simulink model "DRLHevIps"  (R2025b)
settings: Solver=ode23tb  StartTime=0  StopTime=stop_time+1  FixedStep=ts  RelTol=1e-3  AbsTol=1e-4
model workspace (MAT data in the model file):
  BattChrgMax : Simulink.Parameter (value not decoded)
  BattDischrgMax : Simulink.Parameter (value not decoded)
  BrkPrsMax : Simulink.Parameter (value not decoded)
  DiffRatio : Simulink.Parameter (value not decoded)
  EVSpdLmt : Simulink.Parameter (value not decoded)
  EngIdle : Simulink.Parameter (value not decoded)
  EngPwr : Simulink.Parameter (value not decoded)
  EngSpd : Simulink.Parameter (value not decoded)
  EngTrq : Simulink.Parameter (value not decoded)
  EngTrqWhl : Simulink.Parameter (value not decoded)
  GenMapEff : Simulink.Parameter (value not decoded)
  GenMapSpdIndex : Simulink.Parameter (value not decoded)
  GenMapTrqIndex : Simulink.Parameter (value not decoded)
  GenPwrMax : Simulink.Parameter (value not decoded)
  GenSpd : Simulink.Parameter (value not decoded)
  GenTrq : Simulink.Parameter (value not decoded)
  GenTrqMax : Simulink.Parameter (value not decoded)
  MotMapEff : Simulink.Parameter (value not decoded)
  MotMapSpdIndex : Simulink.Parameter (value not decoded)
  MotMapTrqIndex : Simulink.Parameter (value not decoded)
  MotPwr : Simulink.Parameter (value not decoded)
  MotSpd : Simulink.Parameter (value not decoded)
  MotTrq : Simulink.Parameter (value not decoded)
  Ndiff : Simulink.Parameter (value not decoded)
  Nr1 : Simulink.Parameter (value not decoded)
  Nr2 : Simulink.Parameter (value not decoded)
  Ns1 : Simulink.Parameter (value not decoded)
  Ns2 : Simulink.Parameter (value not decoded)
  NsysWhl : Simulink.Parameter (value not decoded)
  SOCChrgFactor : Simulink.Parameter (value not decoded)
  SOCerr : Simulink.Parameter (value not decoded)
  SOCmax : Simulink.Parameter (value not decoded)
  SOCmin : Simulink.Parameter (value not decoded)
  SOCtarget : Simulink.Parameter (value not decoded)
  SysTrqWhl : Simulink.Parameter (value not decoded)
  k : Simulink.Parameter (value not decoded)
values from neighbouring files (symbols this model uses):
  cyc_time = WLTC(:,1)    [mdlrun_time_DG.m]
  cyc_vel = WLTC(:,2)    [mdlrun_time_DG.m]
  en_actsmo = 1    [mdlrun_time_DG.m]
  en_elec = 1    [mdlrun_time_DG.m]
  en_gas = 1    [mdlrun_time_DG.m]
  en_SOCpen = 1    [mdlrun_time_DG.m]
  k_actsmo = 5e-2    (= 0.05)    [mdlrun_time_DG.m]
  k_elec = 1    [mdlrun_time_DG.m]
  k_gas = 1    [mdlrun_time_DG.m]
  k_SOCpen = 1.2    [mdlrun_time_DG.m]
  obs_max = 1e4*[0.0020, 0.0090, 0.0100, 0.0100, 8.4000, 0.0100,                0.0056, 0.1011, 2.8000,      0, 0.0001, 0.0132,                0.0740, 2.6065, 0.0339, 0.0949, 0.0117, 2.4444]    [mdlrun_time_DG.m]
  obs_min = 1e4*[0.0010, 0.0070,      0,      0, 0.8400,      0,                     0, -0.0005,     0, -2.8000,     0, -0.0032               -0.0694, -2.7092, -0.0030,    0, -0.0001, -2.7647]    [mdlrun_time_DG.m]
  Price_elec = 1    [mdlrun_time_DG.m]
  Price_gas = 7.14    [mdlrun_time_DG.m]
  rho_gas = 0.739    [mdlrun_time_DG.m]
  stop_time = cyc_time(end)    [mdlrun_time_DG.m]
  ts = 1    [mdlrun_time_DG.m]
symbols that are objects in the model workspace (value not decoded): BattChrgMax, BattDischrgMax, BrkPrsMax, DiffRatio, EngIdle, EngPwr, EngSpd, EngTrq, EngTrqWhl, EVSpdLmt, GenMapSpdIndex, GenMapTrqIndex, GenPwrMax, GenSpd, GenTrq, GenTrqMax, k, MotMapSpdIndex, MotMapTrqIndex, MotPwr, MotSpd, MotTrq, Ndiff, Nr1, Nr2, Ns1, Ns2, NsysWhl, SOCChrgFactor, SOCerr, SOCmin, SOCtarget, SysTrqWhl
undefined symbols (not defined in the file or in its folder): n_ool, T_ool
libraries: simulink x29, autolibutils x6, slpidlib x2, rllib x2, SignalEditorBlockLib x1, autolibshared x1, autolibhevctrlrcommon x1
(part 4 of 4)

== system DRLHevIps/xCU/xCU/VCU/Rule_Based_DataGen/Subsystem ==
  note: 4 brakes*(mu*pi*Ba^2*Rm*Npads/4)*P
  note: T / 4 brakes*(mu*pi*Ba^2*Rm*Npads/4)
  BattSoc : Inport
  VehSpd : Inport  Port=2
  MotSpd : Inport  Port=3
  "BrkPrsReq " : Inport  Port=4
  ChrgLmt : Lookup_n-D  NumberOfTableDimensions=1  BreakpointsForDimension1=[0:10:100]  Table=[1 1 1 1 1 1 1 1 0.7 0.35 0]  ExtrapMethod=Clip  UseLastTableValue=on  InternalRulePriority=Speed  RndMeth=Simplest
  Constant : Constant  Value=4*(0.2*pi*0.05^2*0.1778*2/4)
  Constant1 : Constant  Value=4*(0.2*pi*0.05^2*0.1778*2/4)
  Gain : Gain  Gain=-1
  MaxMotTrqVsSpd : Lookup_n-D  NumberOfTableDimensions=1  BreakpointsForDimension1=MotSpd  Table=MotTrq  ExtrapMethod=Clip  UseLastTableValue=on  InternalRulePriority=Speed  OutDataTypeStr=Inherit: Inherit from 'Table data'  RndMeth=Simplest
  MinMax : MinMax  Inputs=2
  MotTrqReflectedToWheels : Gain  Gain=(Nr2/Ns2)*Ndiff
  Negative 5 : Saturate  UpperLimit=inf  LowerLimit=0
  Product1 : Product
  Product2 : Product
  Product3 : Product
  Product4 : Product  Inputs=*/
  RegenBrakingCutoff : Lookup_n-D  NumberOfTableDimensions=1  BreakpointsForDimension1=[2.2 4.5]  Table=[0 1]  ExtrapMethod=Clip  UseLastTableValue=on  InternalRulePriority=Speed  RndMeth=Simplest
  Subtract : Sum  Inputs=+-
  WhlTrqReflectedToMot : Gain  Gain=1/((Nr2/Ns2)*Ndiff)
  rads_to_rpm : Gain  Gain=30/pi
  " MotTrqCmdRegen" : Outport  VectorParamsAs1DForOutWhenUnconnected=off
  " BrkCmd" : Outport  Port=2  VectorParamsAs1DForOutWhenUnconnected=off
  wires:
  VehSpd/1 -> RegenBrakingCutoff/1
  Subtract/1 -> Negative 5/1
  Product4/1 -> " BrkCmd"/1
  RegenBrakingCutoff/1 -> Product1/1
  "BrkPrsReq "/1 -> Product2/1  "BrkPrsReq"
  Negative 5/1 -> Product4/1  "BrkTrqFric"
  MaxMotTrqVsSpd/1 -> MotTrqReflectedToWheels/1  "MotTrqMax"
  MotSpd/1 -> rads_to_rpm/1
  MinMax/1 -> Product3/1  "min"
  Product2/1 -> MinMax/1, Subtract/1  "BrkTrqReqTotal"
  rads_to_rpm/1 -> MaxMotTrqVsSpd/1
  Gain/1 -> " MotTrqCmdRegen"/1  "MotTrqCmdRegen"
  Product1/1 -> Product3/2  "RegenFactor"
  Product3/1 -> WhlTrqReflectedToMot/1, Subtract/2  "MotTrqRegenWhl"
  WhlTrqReflectedToMot/1 -> Gain/1
  ChrgLmt/1 -> Product1/2
  BattSoc/1 -> ChrgLmt/1
  Constant/1 -> Product2/2
  MotTrqReflectedToWheels/1 -> MinMax/2  "MotTrqMaxWhls"
  Constant1/1 -> Product4/2

== system DRLHevIps/xCU/xCU/VCU/DRL_Based2_0/Motor Torque Arbitration and Power Management/Power Management ==
  BattPwrDischrgLmt : Inport
  GenPwrElec : Inport  Port=2
  BattPwrChrgLmt : Inport  Port=3
  MotSpd : Inport  Port=4
  MotTrqCmd : Inport  Port=5
  Check Within Limits : Subsystem
  ElecToMechPwr : Product  Inputs=*/
  Mech to Elec Power Estimate : Subsystem
  MechPwrToTrq : Product  Inputs=*/
  Saturation1 : Saturate  UpperLimit=inf  LowerLimit=0
  Saturation2 : Saturate  UpperLimit=0  LowerLimit=-inf
  Sum : Sum  Inputs=+-
  Sum4 : Sum  Inputs=-+
  Switch : Switch  Criteria=u2 > Threshold  SaturateOnIntegerOverflow=off  InputSameDT=off
  Torque Limit : Subsystem
  div0protect - poly : autolibutils/div0protect - poly  thresh=2  ZeroCross1=off  aMode=aMode
  MotTrqLim : Outport  VectorParamsAs1DForOutWhenUnconnected=off
  wires:
  Check Within Limits/1(InLimit) -> Switch/2
  Switch/1 -> Torque Limit/1(MotTrq)
  Check Within Limits/2(y) -> ElecToMechPwr/1
  Saturation2/1 -> Check Within Limits/3(lo)
  Mech to Elec Power Estimate/1(MotPwrElecReq) -> Check Within Limits/2(u)
  Saturation1/1 -> Check Within Limits/1(up)
  Torque Limit/1(MotTrqCmd) -> MotTrqLim/1
  MechPwrToTrq/1 -> Switch/3
  ElecToMechPwr/1 -> MechPwrToTrq/1
  Mech to Elec Power Estimate/2(eff2k) -> ElecToMechPwr/2
  div0protect - poly/1 -> MechPwrToTrq/2
  MotTrqCmd/1 -> Mech to Elec Power Estimate/1(MotTrqCmd), Switch/1
  MotSpd/1 -> Mech to Elec Power Estimate/2(MotSpd), div0protect - poly/1, Torque Limit/2(MotSpd)
  BattPwrDischrgLmt/1 -> Sum/1
  GenPwrElec/1 -> Sum4/1, Sum/2
  Sum/1 -> Saturation1/1
  Sum4/1 -> Saturation2/1
  BattPwrChrgLmt/1 -> Sum4/2

== system DRLHevIps/xCU/xCU/VCU/Rule_Based/Motor Torque Arbitration and Power Management/Power Management ==
  BattPwrDischrgLmt : Inport
  GenPwrElec : Inport  Port=2
  BattPwrChrgLmt : Inport  Port=3
  MotSpd : Inport  Port=4
  MotTrqCmd : Inport  Port=5
  Check Within Limits : Subsystem
  ElecToMechPwr : Product  Inputs=*/
  Mech to Elec Power Estimate : Subsystem
  MechPwrToTrq : Product  Inputs=*/
  Saturation1 : Saturate  UpperLimit=inf  LowerLimit=0
  Saturation2 : Saturate  UpperLimit=0  LowerLimit=-inf
  Sum : Sum  Inputs=+-
  Sum4 : Sum  Inputs=-+
  Switch : Switch  Criteria=u2 > Threshold  SaturateOnIntegerOverflow=off  InputSameDT=off
  Torque Limit : Subsystem
  div0protect - poly : autolibutils/div0protect - poly  thresh=2  ZeroCross1=off  aMode=aMode
  MotTrqLim : Outport  VectorParamsAs1DForOutWhenUnconnected=off
  wires:
  BattPwrChrgLmt/1 -> Sum4/2
  Sum4/1 -> Saturation2/1
  Sum/1 -> Saturation1/1
  GenPwrElec/1 -> Sum/2, Sum4/1
  BattPwrDischrgLmt/1 -> Sum/1
  MotSpd/1 -> Torque Limit/2(MotSpd), div0protect - poly/1, Mech to Elec Power Estimate/2(MotSpd)
  MotTrqCmd/1 -> Switch/1, Mech to Elec Power Estimate/1(MotTrqCmd)
  div0protect - poly/1 -> MechPwrToTrq/2
  Mech to Elec Power Estimate/2(eff2k) -> ElecToMechPwr/2
  ElecToMechPwr/1 -> MechPwrToTrq/1
  MechPwrToTrq/1 -> Switch/3
  Torque Limit/1(MotTrqCmd) -> MotTrqLim/1
  Saturation1/1 -> Check Within Limits/1(up)
  Mech to Elec Power Estimate/1(MotPwrElecReq) -> Check Within Limits/2(u)
  Saturation2/1 -> Check Within Limits/3(lo)
  Check Within Limits/2(y) -> ElecToMechPwr/1
  Switch/1 -> Torque Limit/1(MotTrq)
  Check Within Limits/1(InLimit) -> Switch/2

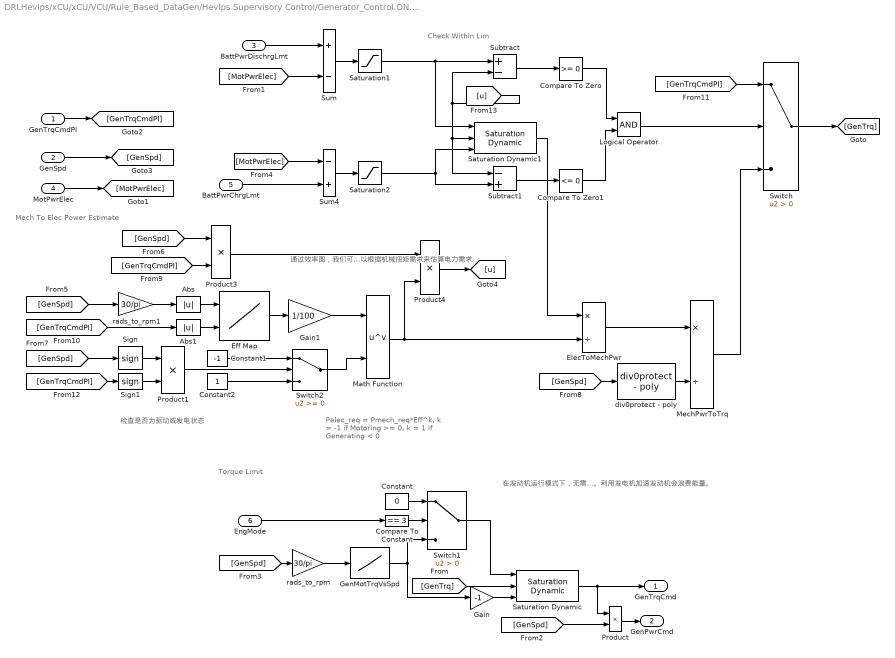
== system DRLHevIps/xCU/xCU/VCU/Rule_Based_DataGen/HevIps Supervisory Control/Generator_Control.ON.GenControl/Power Management ==
  note: Check Within Lim
  note: Mech To Elec Power Estimate
  note: Torque Limit
  note: 在发动机运行模式下，无需保持发电机扭矩大于零，因为发电机通过制动发动机来维持所需速度。利用发电机加速发动机会浪费能量。
  note: 检查是否为驱动或发电状态
  note: 通过效率图，我们可以根据机械扭矩需求来估算电力需求。
  note: Pelec_req = Pmech_req*Eff^k,
      | k = -1 if Motoring >= 0,
      | k = 1 if Generating < 0
  GenTrqCmdPI : Inport
  GenSpd : Inport  Port=2
  BattPwrDischrgLmt : Inport  Port=3
  MotPwrElec : Inport  Port=4
  BattPwrChrgLmt : Inport  Port=5
  EngMode : Inport  Port=6
  Abs : Abs  SaturateOnIntegerOverflow=off
  Abs1 : Abs  SaturateOnIntegerOverflow=off
  Compare To Constant : simulink/Logic and Bit Operations/Compare To Constant  relop===  const=3  OutDataTypeStr=boolean
  Compare To Zero : simulink/Logic and Bit Operations/Compare To Zero  relop=>=  OutDataTypeStr=boolean
  Compare To Zero1 : simulink/Logic and Bit Operations/Compare To Zero  relop=<=  OutDataTypeStr=boolean
  Constant : Constant  Value=0
  Constant1 : Constant  Value=-1  SampleTime=-1
  Constant2 : Constant  SampleTime=-1
  Eff Map : Lookup_n-D  BreakpointsForDimension1=GenMapSpdIndex  BreakpointsForDimension2=GenMapTrqIndex  Table=GenMapEff'  ExtrapMethod=Clip  UseLastTableValue=on  InternalRulePriority=Speed  OutDataTypeStr=Inherit: Inherit from 'Table data'  RndMeth=Simplest
      settings: InputPortMap=u0,u1
  ElecToMechPwr : Product  Inputs=*/
  Gain : Gain  Gain=-1
  Gain1 : Gain  Gain=1/100
  GenMotTrqVsSpd : Lookup_n-D  NumberOfTableDimensions=1  BreakpointsForDimension1=GenSpd  Table=GenTrq  ExtrapMethod=Clip  UseLastTableValue=on  InternalRulePriority=Speed  OutDataTypeStr=Inherit: Inherit from 'Table data'  RndMeth=Simplest
  Logical Operator : Logic  AllPortsSameDT=off  OutDataTypeStr=boolean
  Math Function : Math  Operator=pow  SignedPower=on  OutputSignalType=real
  MechPwrToTrq : Product  Inputs=*/
  Product{,1,3..4} (4 alike) : Product
  Saturation Dynamic : simulink/Discontinuities/Saturation Dynamic  OutMin=[]  OutMax=[]  OutDataTypeStr=Inherit: Same as second input  OutDataType=fixdt(1, 16)  OutScaling=2^-10  DoSatur=off
  Saturation Dynamic1 : simulink/Discontinuities/Saturation Dynamic  OutMin=[]  OutMax=[]  OutDataTypeStr=Inherit: Same as second input  OutDataType=fixdt(1, 16)  OutScaling=2^-10  DoSatur=off
  Saturation1 : Saturate  UpperLimit=inf  LowerLimit=0
  Saturation2 : Saturate  UpperLimit=0  LowerLimit=-inf
  Sign : Signum
  Sign1 : Signum
  Subtract : Sum  Inputs=+-
  Subtract1 : Sum  Inputs=-+
  Sum : Sum  Inputs=+-
  Sum4 : Sum  Inputs=-+
  Switch : Switch  Criteria=u2 > Threshold  SaturateOnIntegerOverflow=off  InputSameDT=off
  Switch1 : Switch  Criteria=u2 > Threshold  SaturateOnIntegerOverflow=off  InputSameDT=off
  Switch2 : Switch  SaturateOnIntegerOverflow=off  InputSameDT=off
  div0protect - poly : autolibutils/div0protect - poly  thresh=2  ZeroCross1=off  aMode=aMode
  rads_to_rpm : Gain  Gain=30/pi
  rads_to_rpm1 : Gain  Gain=30/pi
  GenTrqCmd : Outport  VectorParamsAs1DForOutWhenUnconnected=off
  GenPwrCmd : Outport  Port=2  VectorParamsAs1DForOutWhenUnconnected=off
  wires:
  Logical Operator/1 -> Switch/2
  Switch/1 -> [GenTrq]
  Product/1 -> GenPwrCmd/1
  MechPwrToTrq/1 -> Switch/3
  Saturation Dynamic/1 -> Product/1, GenTrqCmd/1
  Math Function/1 -> Product4/2, ElecToMechPwr/2
  Saturation Dynamic1/1 -> ElecToMechPwr/1
  div0protect - poly/1 -> MechPwrToTrq/2
  ElecToMechPwr/1 -> MechPwrToTrq/1
  BattPwrDischrgLmt/1 -> Sum/1
  MotPwrElec/1 -> [MotPwrElec]
  Sum/1 -> Saturation1/1
  Sum4/1 -> Saturation2/1
  BattPwrChrgLmt/1 -> Sum4/2
  [GenSpd] -> Product/2
  rads_to_rpm/1 -> GenMotTrqVsSpd/1
  Constant/1 -> Switch1/1
  GenMotTrqVsSpd/1 -> Gain/1, Switch1/3
  Gain/1 -> Saturation Dynamic/3
  [GenTrq] -> Saturation Dynamic/2
  [GenSpd] -> rads_to_rpm/1
  EngMode/1 -> Compare To Constant/1
  Compare To Constant/1 -> Switch1/2
  Switch1/1 -> Saturation Dynamic/1
  Product3/1 -> Product4/1
  Switch2/1 -> Math Function/2
  Constant1/1 -> Switch2/1
  Constant2/1 -> Switch2/3
  Eff Map/1 -> Gain1/1
  GenTrqCmdPI/1 -> [GenTrqCmdPI]
  Abs/1 -> Eff Map/1
  Gain1/1 -> Math Function/1
  Abs1/1 -> Eff Map/2
  rads_to_rpm1/1 -> Abs/1
  Product1/1 -> Switch2/2
  Sign/1 -> Product1/1
  Sign1/1 -> Product1/2
  GenSpd/1 -> [GenSpd]
  [MotPwrElec] -> Sum/2
  [MotPwrElec] -> Sum4/1
  [GenSpd] -> Product3/1
  [GenSpd] -> rads_to_rpm1/1
  [GenSpd] -> Sign/1
  [GenSpd] -> div0protect - poly/1
  [GenTrqCmdPI] -> Product3/2
  [GenTrqCmdPI] -> Abs1/1
  [GenTrqCmdPI] -> Switch/1
  [GenTrqCmdPI] -> Sign1/1
  Product4/1 -> [u]
  Saturation2/1 -> Subtract1/2, Saturation Dynamic1/3
  Saturation1/1 -> Subtract/1, Saturation Dynamic1/1
  [u] -> Saturation Dynamic1/2, Subtract1/1, Subtract/2
  Subtract/1 -> Compare To Zero/1
  Subtract1/1 -> Compare To Zero1/1
  Compare To Zero/1 -> Logical Operator/1
  Compare To Zero1/1 -> Logical Operator/2

== system DRLHevIps/xCU/xCU/VCU/Rule_Based_DataGen/Motor Torque Arbitration and Power Management/Power Management ==
  BattPwrDischrgLmt : Inport
  GenPwrElec : Inport  Port=2
  BattPwrChrgLmt : Inport  Port=3
  MotSpd : Inport  Port=4
  MotTrqCmd : Inport  Port=5
  Check Within Limits : Subsystem
  ElecToMechPwr : Product  Inputs=*/
  Mech to Elec Power Estimate : Subsystem
  MechPwrToTrq : Product  Inputs=*/
  Saturation1 : Saturate  UpperLimit=inf  LowerLimit=0
  Saturation2 : Saturate  UpperLimit=0  LowerLimit=-inf
  Sum : Sum  Inputs=+-
  Sum4 : Sum  Inputs=-+
  Switch : Switch  Criteria=u2 > Threshold  SaturateOnIntegerOverflow=off  InputSameDT=off
  Torque Limit : Subsystem
  div0protect - poly : autolibutils/div0protect - poly  thresh=2  ZeroCross1=off  aMode=aMode
  MotTrqLim : Outport  VectorParamsAs1DForOutWhenUnconnected=off
  wires:
  BattPwrChrgLmt/1 -> Sum4/2
  Sum4/1 -> Saturation2/1
  Sum/1 -> Saturation1/1
  GenPwrElec/1 -> Sum/2, Sum4/1
  BattPwrDischrgLmt/1 -> Sum/1
  MotSpd/1 -> Torque Limit/2(MotSpd), div0protect - poly/1, Mech to Elec Power Estimate/2(MotSpd)
  MotTrqCmd/1 -> Switch/1, Mech to Elec Power Estimate/1(MotTrqCmd)
  div0protect - poly/1 -> MechPwrToTrq/2
  Mech to Elec Power Estimate/2(eff2k) -> ElecToMechPwr/2
  ElecToMechPwr/1 -> MechPwrToTrq/1
  MechPwrToTrq/1 -> Switch/3
  Torque Limit/1(MotTrqCmd) -> MotTrqLim/1
  Saturation1/1 -> Check Within Limits/1(up)
  Mech to Elec Power Estimate/1(MotPwrElecReq) -> Check Within Limits/2(u)
  Saturation2/1 -> Check Within Limits/3(lo)
  Check Within Limits/2(y) -> ElecToMechPwr/1
  Switch/1 -> Torque Limit/1(MotTrq)
  Check Within Limits/1(InLimit) -> Switch/2

== system DRLHevIps/xCU/xCU/VCU/DRL_Based2_0/Motor Torque Arbitration and Power Management/Power Management/Check Within Limits ==
  up : Inport
  u : Inport  Port=2
  lo : Inport  Port=3
  Compare To Zero : simulink/Logic and Bit Operations/Compare To Zero  relop=>=  OutDataTypeStr=boolean
  Compare To Zero1 : simulink/Logic and Bit Operations/Compare To Zero  relop=<=  OutDataTypeStr=boolean
  Logical Operator : Logic  AllPortsSameDT=off  OutDataTypeStr=boolean
  Saturation Dynamic1 : simulink/Discontinuities/Saturation Dynamic  OutMin=[]  OutMax=[]  OutDataTypeStr=Inherit: Same as second input  OutDataType=fixdt(1, 16)  OutScaling=2^-10  DoSatur=off
  Subtract : Sum  Inputs=+-
  Subtract1 : Sum  Inputs=-+
  InLimit : Outport  VectorParamsAs1DForOutWhenUnconnected=off
  y : Outport  Port=2  VectorParamsAs1DForOutWhenUnconnected=off
  wires:
  Logical Operator/1 -> InLimit/1
  Compare To Zero1/1 -> Logical Operator/2
  Compare To Zero/1 -> Logical Operator/1
  Subtract1/1 -> Compare To Zero1/1
  Subtract/1 -> Compare To Zero/1
  u/1 -> Saturation Dynamic1/2, Subtract/2, Subtract1/1
  up/1 -> Saturation Dynamic1/1, Subtract/1
  lo/1 -> Saturation Dynamic1/3, Subtract1/2
  Saturation Dynamic1/1 -> y/1

== system DRLHevIps/xCU/xCU/VCU/DRL_Based2_0/Motor Torque Arbitration and Power Management/Power Management/Mech to Elec Power Estimate ==
  note: Pelec_req = Pmech_req*Eff^k,
      | k = -1 if Motoring >= 0,
      | k = 1 if Generating < 0
  note: Using an Efficiency Map, we can estimate the
      | Electric Power from the Mechanical  Torque Request.
  note: Check if Motoring
      | or Generating
  MotTrqCmd : Inport
  MotSpd : Inport  Port=2
  Abs : Abs  SaturateOnIntegerOverflow=off
  Abs1 : Abs  SaturateOnIntegerOverflow=off
  Constant1 : Constant  Value=-1  SampleTime=-1
  Constant2 : Constant  SampleTime=-1
  Eff Map : Lookup_n-D  BreakpointsForDimension1=MotMapSpdIndex  BreakpointsForDimension2=MotMapTrqIndex  Table=MotMapEff'  ExtrapMethod=Clip  UseLastTableValue=on  InternalRulePriority=Speed  OutDataTypeStr=Inherit: Inherit from 'Table data'  RndMeth=Simplest
      settings: InputPortMap=u0,u1
  Gain1 : Gain  Gain=1/100
  Math Function : Math  Operator=pow  SignedPower=on  OutputSignalType=real
  Product : Product
  Product3 : Product
  Product4 : Product
  Sign : Signum
  Sign1 : Signum
  Switch2 : Switch  SaturateOnIntegerOverflow=off  InputSameDT=off
  rads_to_rpm : Gain  Gain=30/pi
  MotPwrElecReq : Outport  VectorParamsAs1DForOutWhenUnconnected=off
  eff2k : Outport  Port=2  VectorParamsAs1DForOutWhenUnconnected=off
  wires:
  MotSpd/1 -> Sign/1, rads_to_rpm/1, Product3/1
  Sign1/1 -> Product/2
  Sign/1 -> Product/1
  Product/1 -> Switch2/2
  rads_to_rpm/1 -> Abs/1
  Abs1/1 -> Eff Map/2
  Product4/1 -> MotPwrElecReq/1
  Math Function/1 -> Product4/2, eff2k/1
  Gain1/1 -> Math Function/1
  Abs/1 -> Eff Map/1
  MotTrqCmd/1 -> Sign1/1, Abs1/1, Product3/2
  Eff Map/1 -> Gain1/1
  Constant2/1 -> Switch2/3
  Constant1/1 -> Switch2/1
  Switch2/1 -> Math Function/2
  Product3/1 -> Product4/1

== system DRLHevIps/xCU/xCU/VCU/DRL_Based2_0/Motor Torque Arbitration and Power Management/Power Management/Torque Limit ==
  MotTrq : Inport
  MotSpd : Inport  Port=2
  Gain : Gain  Gain=-1
  MaxMotTrqVsSpd : Lookup_n-D  NumberOfTableDimensions=1  BreakpointsForDimension1=MotSpd  Table=MotTrq  ExtrapMethod=Clip  UseLastTableValue=on  InternalRulePriority=Speed  OutDataTypeStr=Inherit: Inherit from 'Table data'  RndMeth=Simplest
  Saturation Dynamic : simulink/Discontinuities/Saturation Dynamic  OutMin=[]  OutMax=[]  OutDataTypeStr=Inherit: Same as second input  OutDataType=fixdt(1, 16)  OutScaling=2^-10  DoSatur=off
  rads_to_rpm : Gain  Gain=30/pi
  MotTrqCmd : Outport  VectorParamsAs1DForOutWhenUnconnected=off
  wires:
  Gain/1 -> Saturation Dynamic/3
  rads_to_rpm/1 -> MaxMotTrqVsSpd/1
  MaxMotTrqVsSpd/1 -> Saturation Dynamic/1, Gain/1
  MotSpd/1 -> rads_to_rpm/1
  Saturation Dynamic/1 -> MotTrqCmd/1
  MotTrq/1 -> Saturation Dynamic/2

== system DRLHevIps/xCU/xCU/VCU/Rule_Based/Motor Torque Arbitration and Power Management/Power Management/Check Within Limits ==
  up : Inport
  u : Inport  Port=2
  lo : Inport  Port=3
  Compare To Zero : simulink/Logic and Bit Operations/Compare To Zero  relop=>=  OutDataTypeStr=boolean
  Compare To Zero1 : simulink/Logic and Bit Operations/Compare To Zero  relop=<=  OutDataTypeStr=boolean
  Logical Operator : Logic  AllPortsSameDT=off  OutDataTypeStr=boolean
  Saturation Dynamic1 : simulink/Discontinuities/Saturation Dynamic  OutMin=[]  OutMax=[]  OutDataTypeStr=Inherit: Same as second input  OutDataType=fixdt(1, 16)  OutScaling=2^-10  DoSatur=off
  Subtract : Sum  Inputs=+-
  Subtract1 : Sum  Inputs=-+
  InLimit : Outport  VectorParamsAs1DForOutWhenUnconnected=off
  y : Outport  Port=2  VectorParamsAs1DForOutWhenUnconnected=off
  wires:
  Saturation Dynamic1/1 -> y/1
  lo/1 -> Subtract1/2, Saturation Dynamic1/3
  up/1 -> Subtract/1, Saturation Dynamic1/1
  u/1 -> Subtract1/1, Subtract/2, Saturation Dynamic1/2
  Subtract/1 -> Compare To Zero/1
  Subtract1/1 -> Compare To Zero1/1
  Compare To Zero/1 -> Logical Operator/1
  Compare To Zero1/1 -> Logical Operator/2
  Logical Operator/1 -> InLimit/1

== system DRLHevIps/xCU/xCU/VCU/Rule_Based/Motor Torque Arbitration and Power Management/Power Management/Mech to Elec Power Estimate ==
  note: Check if Motoring
      | or Generating
  note: Using an Efficiency Map, we can estimate the
      | Electric Power from the Mechanical  Torque Request.
  note: Pelec_req = Pmech_req*Eff^k,
      | k = -1 if Motoring >= 0,
      | k = 1 if Generating < 0
  MotTrqCmd : Inport
  MotSpd : Inport  Port=2
  Abs : Abs  SaturateOnIntegerOverflow=off
  Abs1 : Abs  SaturateOnIntegerOverflow=off
  Constant1 : Constant  Value=-1  SampleTime=-1
  Constant2 : Constant  SampleTime=-1
  Eff Map : Lookup_n-D  BreakpointsForDimension1=MotMapSpdIndex  BreakpointsForDimension2=MotMapTrqIndex  Table=MotMapEff'  ExtrapMethod=Clip  UseLastTableValue=on  InternalRulePriority=Speed  OutDataTypeStr=Inherit: Inherit from 'Table data'  RndMeth=Simplest
      settings: InputPortMap=u0,u1
  Gain1 : Gain  Gain=1/100
  Math Function : Math  Operator=pow  SignedPower=on  OutputSignalType=real
  Product : Product
  Product3 : Product
  Product4 : Product
  Sign : Signum
  Sign1 : Signum
  Switch2 : Switch  SaturateOnIntegerOverflow=off  InputSameDT=off
  rads_to_rpm : Gain  Gain=30/pi
  MotPwrElecReq : Outport  VectorParamsAs1DForOutWhenUnconnected=off
  eff2k : Outport  Port=2  VectorParamsAs1DForOutWhenUnconnected=off
  wires:
  Product3/1 -> Product4/1
  Switch2/1 -> Math Function/2
  Constant1/1 -> Switch2/1
  Constant2/1 -> Switch2/3
  Eff Map/1 -> Gain1/1
  MotTrqCmd/1 -> Product3/2, Abs1/1, Sign1/1
  Abs/1 -> Eff Map/1
  Gain1/1 -> Math Function/1
  Math Function/1 -> eff2k/1, Product4/2
  Product4/1 -> MotPwrElecReq/1
  Abs1/1 -> Eff Map/2
  rads_to_rpm/1 -> Abs/1
  Product/1 -> Switch2/2
  Sign/1 -> Product/1
  Sign1/1 -> Product/2
  MotSpd/1 -> Product3/1, rads_to_rpm/1, Sign/1

== system DRLHevIps/xCU/xCU/VCU/Rule_Based/Motor Torque Arbitration and Power Management/Power Management/Torque Limit ==
  MotTrq : Inport
  MotSpd : Inport  Port=2
  Gain : Gain  Gain=-1
  MaxMotTrqVsSpd : Lookup_n-D  NumberOfTableDimensions=1  BreakpointsForDimension1=MotSpd  Table=MotTrq  ExtrapMethod=Clip  UseLastTableValue=on  InternalRulePriority=Speed  OutDataTypeStr=Inherit: Inherit from 'Table data'  RndMeth=Simplest
  Saturation Dynamic : simulink/Discontinuities/Saturation Dynamic  OutMin=[]  OutMax=[]  OutDataTypeStr=Inherit: Same as second input  OutDataType=fixdt(1, 16)  OutScaling=2^-10  DoSatur=off
  rads_to_rpm : Gain  Gain=30/pi
  MotTrqCmd : Outport  VectorParamsAs1DForOutWhenUnconnected=off
  wires:
  MotTrq/1 -> Saturation Dynamic/2
  Saturation Dynamic/1 -> MotTrqCmd/1
  MotSpd/1 -> rads_to_rpm/1
  MaxMotTrqVsSpd/1 -> Gain/1, Saturation Dynamic/1
  rads_to_rpm/1 -> MaxMotTrqVsSpd/1
  Gain/1 -> Saturation Dynamic/3

== system DRLHevIps/xCU/xCU/VCU/Rule_Based_DataGen/Motor Torque Arbitration and Power Management/Power Management/Check Within Limits ==
  up : Inport
  u : Inport  Port=2
  lo : Inport  Port=3
  Compare To Zero : simulink/Logic and Bit Operations/Compare To Zero  relop=>=  OutDataTypeStr=boolean
  Compare To Zero1 : simulink/Logic and Bit Operations/Compare To Zero  relop=<=  OutDataTypeStr=boolean
  Logical Operator : Logic  AllPortsSameDT=off  OutDataTypeStr=boolean
  Saturation Dynamic1 : simulink/Discontinuities/Saturation Dynamic  OutMin=[]  OutMax=[]  OutDataTypeStr=Inherit: Same as second input  OutDataType=fixdt(1, 16)  OutScaling=2^-10  DoSatur=off
  Subtract : Sum  Inputs=+-
  Subtract1 : Sum  Inputs=-+
  InLimit : Outport  VectorParamsAs1DForOutWhenUnconnected=off
  y : Outport  Port=2  VectorParamsAs1DForOutWhenUnconnected=off
  wires:
  Saturation Dynamic1/1 -> y/1
  lo/1 -> Subtract1/2, Saturation Dynamic1/3
  up/1 -> Subtract/1, Saturation Dynamic1/1
  u/1 -> Subtract1/1, Subtract/2, Saturation Dynamic1/2
  Subtract/1 -> Compare To Zero/1
  Subtract1/1 -> Compare To Zero1/1
  Compare To Zero/1 -> Logical Operator/1
  Compare To Zero1/1 -> Logical Operator/2
  Logical Operator/1 -> InLimit/1

== system DRLHevIps/xCU/xCU/VCU/Rule_Based_DataGen/Motor Torque Arbitration and Power Management/Power Management/Mech to Elec Power Estimate ==
  note: Check if Motoring
      | or Generating
  note: Using an Efficiency Map, we can estimate the
      | Electric Power from the Mechanical  Torque Request.
  note: Pelec_req = Pmech_req*Eff^k,
      | k = -1 if Motoring >= 0,
      | k = 1 if Generating < 0
  MotTrqCmd : Inport
  MotSpd : Inport  Port=2
  Abs : Abs  SaturateOnIntegerOverflow=off
  Abs1 : Abs  SaturateOnIntegerOverflow=off
  Constant1 : Constant  Value=-1  SampleTime=-1
  Constant2 : Constant  SampleTime=-1
  Eff Map : Lookup_n-D  BreakpointsForDimension1=MotMapSpdIndex  BreakpointsForDimension2=MotMapTrqIndex  Table=MotMapEff'  ExtrapMethod=Clip  UseLastTableValue=on  InternalRulePriority=Speed  OutDataTypeStr=Inherit: Inherit from 'Table data'  RndMeth=Simplest
      settings: InputPortMap=u0,u1
  Gain1 : Gain  Gain=1/100
  Math Function : Math  Operator=pow  SignedPower=on  OutputSignalType=real
  Product : Product
  Product3 : Product
  Product4 : Product
  Sign : Signum
  Sign1 : Signum
  Switch2 : Switch  SaturateOnIntegerOverflow=off  InputSameDT=off
  rads_to_rpm : Gain  Gain=30/pi
  MotPwrElecReq : Outport  VectorParamsAs1DForOutWhenUnconnected=off
  eff2k : Outport  Port=2  VectorParamsAs1DForOutWhenUnconnected=off
  wires:
  Product3/1 -> Product4/1
  Switch2/1 -> Math Function/2
  Constant1/1 -> Switch2/1
  Constant2/1 -> Switch2/3
  Eff Map/1 -> Gain1/1
  MotTrqCmd/1 -> Product3/2, Abs1/1, Sign1/1
  Abs/1 -> Eff Map/1
  Gain1/1 -> Math Function/1
  Math Function/1 -> eff2k/1, Product4/2
  Product4/1 -> MotPwrElecReq/1
  Abs1/1 -> Eff Map/2
  rads_to_rpm/1 -> Abs/1
  Product/1 -> Switch2/2
  Sign/1 -> Product/1
  Sign1/1 -> Product/2
  MotSpd/1 -> Product3/1, rads_to_rpm/1, Sign/1

== system DRLHevIps/xCU/xCU/VCU/Rule_Based_DataGen/Motor Torque Arbitration and Power Management/Power Management/Torque Limit ==
  MotTrq : Inport
  MotSpd : Inport  Port=2
  Gain : Gain  Gain=-1
  MaxMotTrqVsSpd : Lookup_n-D  NumberOfTableDimensions=1  BreakpointsForDimension1=MotSpd  Table=MotTrq  ExtrapMethod=Clip  UseLastTableValue=on  InternalRulePriority=Speed  OutDataTypeStr=Inherit: Inherit from 'Table data'  RndMeth=Simplest
  Saturation Dynamic : simulink/Discontinuities/Saturation Dynamic  OutMin=[]  OutMax=[]  OutDataTypeStr=Inherit: Same as second input  OutDataType=fixdt(1, 16)  OutScaling=2^-10  DoSatur=off
  rads_to_rpm : Gain  Gain=30/pi
  MotTrqCmd : Outport  VectorParamsAs1DForOutWhenUnconnected=off
  wires:
  MotTrq/1 -> Saturation Dynamic/2
  Saturation Dynamic/1 -> MotTrqCmd/1
  MotSpd/1 -> rads_to_rpm/1
  MaxMotTrqVsSpd/1 -> Gain/1, Saturation Dynamic/1
  rads_to_rpm/1 -> MaxMotTrqVsSpd/1
  Gain/1 -> Saturation Dynamic/3

== stateflow chart DRLHevIps/xCU/xCU/VCU/Rule_Based_DataGen/HevIps Supervisory Control ==
  settings: enableNonTerminalStates=1
  state Operating_Modes [parallel]
    entry, during:
    WhlPwrCmd = WhlTrqCmd*WhlSpd;
    SOCopt = (SOCtarget/100) - 0.5*VehMass*VehSpd*VehSpd*EffRechrg/BattEnergy;
    ChrgPwr = SOCChrgFactor*(SOCopt - SOC/100)*AccelPed;
    EngOnReq = EngOnCalc(SOC,BattPwr,BattPwrDischrgLmt,VehSpd,EVSpdLmt,AccelPed,WhlPwrCmd,SOCopt,OpMode);
    settings: executionOrder=1
    state Driving
      state EV
        entry, during:
        OpMode = 1;
        EngPwrCmd = 0;
        MotMode = 1;
      state Wait
        entry, during:
        OpMode = 2;
        MotMode = 1;
      state HEV
        entry:
        InitFlag = 1;
        MotMode = 2;
        during:
        [Low,High] = ModeSelection(WhlSpd,WhlPwrCmd,AccelPed,ChrgPwr,BattPwrChrgLmt);
        exit:
        EngPwrCmd = 0;
        MotPwrCmd = 0;
        MotMode = 1;
        state Low_Power_Charge_Sustain
          entry:
          StateChange = 0;
          during:
          OpMode = 3;
          [EngPwrCmd,MotPwrCmd] = OpMode3(WhlPwrCmd,ChrgPwr,BattPwrChrgLmt,GenPwrCmd,EngTrqOut,EngSpd);
          state [EngPwrCmd,MotPwrCmd] = OpMode3(WhlPwrCmd,ChrgPwr,BattPwrChrgLmt,GenPwrCmd,EngTrqOut,EngSpd) [function]
        state Wait1
          entry:
          StateChange = 1;
        state Wait
          entry:
          StateChange = 1;
        state High_Power_Charge_Deplete
          entry:
          InitFlag = 0;
          StateChange = 0;
          during:
          OpMode = 4;
          [EngPwrCmd,MotPwrCmd] = OpMode4(WhlTrqCmd,WhlSpd,WhlPwrCmd,EngTrqOut);
          state [EngPwrCmd,MotPwrCmd] = OpMode4(WhlTrqCmd,WhlSpd,WhlPwrCmd,EngTrqOut) [function]
        state [Low,High] = ModeSelection(WhlSpd,WhlPwrCmd,AccelPed,ChrgPwr,BattPwrChrgLmt) [function]
        (default) -> Low_Power_Charge_Sustain
        Low_Power_Charge_Sustain -> High_Power_Charge_Deplete [order 1] : [High && InitFlag == 1 ]
        Low_Power_Charge_Sustain -> Operating_Modes.Driving.HEV.Wait [order 2] : [High && InitFlag == 0]
        Operating_Modes.Driving.HEV.Wait1 -> Low_Power_Charge_Sustain : [after(Ts,sec)]
        Operating_Modes.Driving.HEV.Wait -> High_Power_Charge_Deplete : [after(Ts,sec)]
        High_Power_Charge_Deplete -> Operating_Modes.Driving.HEV.Wait1 : [Low]
      (default) -> EV
      EV -> Operating_Modes.Driving.Wait : [EngOnReq]
      Operating_Modes.Driving.Wait -> HEV [order 1] : [EngMode == 3]
      Operating_Modes.Driving.Wait -> EV [order 2] : [~EngOnReq]
      HEV -> EV : [~EngOnReq && EngMode == 1]
    state Wait1
      exit:
      StateChange = 1;
    state Stationary
      entry, during:
      Park = 1;
      exit:
      Park = 0;
      state Charging
        entry, during:
        OpMode =6;
        EngPwrCmd = ChargePowerCalc(SOC);
        exit:
        EngPwrCmd = 0;
        state EngPwrCmd = ChargePowerCalc(SOC) [function]
      state No_Charge
        entry, during:
        OpMode = 5;
      (default) -> No_Charge
      No_Charge -> Charging : [SOC < SOCmin]
      Charging -> No_Charge : [SOC >= SOCtarget]
    state EngOnReq = EngOnCalc(SOC,BattPwr,BattPwrDischrgLmt,VehSpd,EVSpdLmt,AccelPed,WhlPwrCmd,SOCopt,OpMode) [function]
    Driving -> Operating_Modes.Wait1 : [VehSpd < 0.05]
    Operating_Modes.Wait1 -> Driving [order 1] : [AccelPed > 0.1]
    Stationary -> Driving : [AccelPed > 0.01]
    Operating_Modes.Wait1 -> Stationary [order 2] : [after(2, sec)]
    (default) -> Stationary
  state Motor_Control [parallel]
    settings: executionOrder=2
    state Mot_HEV
      entry, during:
      MotTrqCmd = MotTrqHEV(MotPwrCmd,MotSpd);
      state MotTrqCmd = MotTrqHEV(MotPwrCmd,MotSpd) [function]
    state Mot_EV
      entry, during:
      MotTrqCmd = MotTrqEV(WhlTrqCmd);
      state MotTrqCmd = MotTrqEV(WhlTrqCmd) [function]
    (default) -> Mot_EV
    Mot_EV -> Mot_HEV : [MotMode == 2]
    Mot_HEV -> Mot_EV : [MotMode == 1]
  state Generator_Control [parallel]
    settings: executionOrder=3
    state OFF
      entry, during:
      % stay idle // do not start generator control
      EngSpdErr = 0;
      GenTrqCmd = 0;
      GenPwrCmd = 0;
    state wait
    state ON
      entry:
      StateChange = 0;
      during:
      % start and run generator control
      [EngSpdErr,GenTrqCmd,GenPwrCmd] = GenControl(GenSpd,EngSpd,BattPwrDischrgLmt,MotPwrElec,BattPwrChrgLmt,EngSpdCmd,EngMode);
      state [EngSpdErr,GenTrqCmd,GenPwrCmd] = GenControl(GenSpd,EngSpd,BattPwrDischrgLmt,MotPwrElec,BattPwrChrgLmt,EngSpdCmd,EngMode) [function]
    (default) -> OFF
    OFF -> wait : [VehSpd > 0.1 || GenSpd > 10]
    wait -> OFF [order 2] : [VehSpd < 0.05 && GenSpd < 10]
    ON -> OFF [order 1] : [VehSpd < 0.05 && GenSpd < 10]
    wait -> ON [order 1] : [after(Ts,sec)]
    ON -> wait [order 2] : [StateChange == 1]
  state Engine_Control [parallel]
    settings: executionOrder=4
    state Starting
      entry, during:
      StateChange = 0;
      EngMode = 2;
      EngTrqCmd = 0;
      EngSpdCmd = EngIdle;
      exit:
      StateChange = 1;
    state Off
      entry, during:
      EngMode = 1;
      EngTrqCmd = 0;
      EngSpdCmd = 0;
      StateChange = 0;
    state Run
      entry:
      StateChange = 1;
      during:
      StateChange = 0;
      EngMode = 3;
      [EngTrqCmd,EngSpdCmd] = TrqCalc(EngPwrCmd);
      state [EngTrqCmd,EngSpdCmd] = TrqCalc(EngPwrCmd) [function]
    state Wait
    (default) -> Off
    Off -> Starting : [EngOnReq]
    Starting -> Off [order 2] : [~EngOnReq]
    Engine_Control.Wait -> Off [order 2] : [after(1, sec)]
    Starting -> Run [order 1] : [abs(EngSpd - EngIdle) < 5 || EngSpd >= EngIdle]
    Run -> Engine_Control.Wait : [~EngOnReq]
    Engine_Control.Wait -> Run [order 1] : [EngOnReq]
  data: WhlPwrCmd function_input double size=1; ChrgPwr function_input double size=1; BattPwrChrgLmt function_input double size=1; EngPwrCmd function_output; GenPwrCmd function_input double size=1; MotPwrCmd function_output; EngTrqOut function_input double size=1; EngSpd function_input double size=1; WhlTrqCmd function_input double size=1; EngPwrCmd function_output; MotPwrCmd function_output; WhlSpd function_input double size=1; WhlPwrCmd function_input double size=1; EngTrqOut function_input double size=1; Low function_output; High function_output; WhlSpd function_input double size=1; WhlPwrCmd function_input double size=1; AccelPed function_input double size=1; ChrgPwr function_input double size=1; BattPwrChrgLmt function_input double size=1; SOC function_input double size=1; EngPwrCmd function_output; SOC function_input double size=1; EngOnReq function_output; BattPwr function_input double size=1; BattPwrDischrgLmt function_input double size=1; VehSpd function_input double size=1; EVSpdLmt function_input double size=1; AccelPed function_input double size=1; WhlPwrCmd function_input double size=1; SOCopt function_input double size=1; OpMode function_input double size=1; MotPwrCmd function_input double size=1; MotTrqCmd function_output; MotSpd function_input double size=1; WhlTrqCmd function_input double size=1; MotTrqCmd function_output; GenSpd function_input double size=1; EngSpd function_input double size=1; EngSpdErr function_output; GenTrqCmd function_output; GenPwrCmd function_output; BattPwrDischrgLmt function_input double size=1; MotPwrElec function_input double size=1; BattPwrChrgLmt function_input double size=1; EngSpdCmd function_input double size=1; EngMode function_input double size=1; EngPwrCmd function_input double size=1; EngTrqCmd function_output; EngSpdCmd function_output; EVSpdLmt input; EngIdle input; SOCtarget input double =60; SOCmin input [SOCmin..]; SOCChrgFactor input double =150000; SOC input; OpMode output; MotMode output double; EngOnReq output; EngMode output double; EngSpdErr output double; EngPwrCmd output; MotPwrCmd output; EffRechrg constant double =0.6; BattEnergy constant double =4717440; VehMass constant double =1310; ChrgPwr output double; WhlPwrCmd output double; SOCopt output double; VehSpd input; MotSpd input; BattPwrDischrgLmt input; BattPwrChrgLmt input; AccelPed input; EngTrqOut input; GenSpd input; BattPwr input; EngSpd input; WhlTrqCmd input; WhlSpd input; EngSpdCmd output double; GenPwrCmd output double; Park output double; EngTrqCmd output double; GenTrqCmd output double; MotTrqCmd output double; MotPwrElec input; Low local double; High local double; StateChange local double =0; InitFlag local double =0; Ts local double =10e-3

== stateflow chart DRLHevIps/xCU/xCU/VCU/Rule_Based_DataGen/HevIps Supervisory Control/Operating_Modes.EngOnCalc/Timer ==
  state Wait
    du:
    Out = 0;
  state StartTimer
    du:
    Out = 0;
  state TimerDone
    du:
    Out = 1;
  (default) -> StartTimer
  StartTimer -> Wait : [In]
  Wait -> TimerDone [order 2] : after(0.1, sec)
  Wait -> StartTimer [order 1] : [In == 0]
  TimerDone -> StartTimer : [In == 0]
  data: In input; Out output
